simulink model "gm_FFT"  (R2025a)
settings: Solver=VariableStepAuto  StartTime=0.0  StopTime=10.0  RelTol=1e-3
libraries: dsphdlxfrm2 x1
settings Model: Creator=ivanmart  LastModifiedBy=ivanmart
settings OptimizationCC: BlockReduction=off  ConditionallyExecuteInputs=off
settings DebuggingCC: InheritedTsInSrcMsg=none

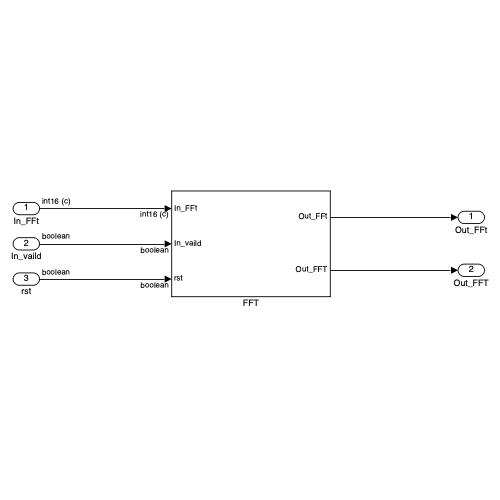
[thumbnail: Simulink's stored preview of the top-level diagram]
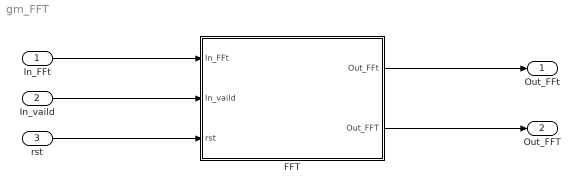
== system gm_FFT ==
  In_FFt : Inport  OutDataTypeStr=fixdt(1,16,0)
      settings: SignalType=complex
  In_vaild : Inport  Port=2  OutDataTypeStr=boolean
  rst : Inport  Port=3  OutDataTypeStr=boolean
  FFT : Subsystem
  Out_FFt : Outport
  Out_FFT : Outport  Port=2
  wires:
  FFT/2(Out_FFT) -> Out_FFT/1
  FFT/1(Out_FFt) -> Out_FFt/1
  rst/1 -> FFT/3(rst)
  In_vaild/1 -> FFT/2(In_vaild)
  In_FFt/1 -> FFT/1(In_FFt)

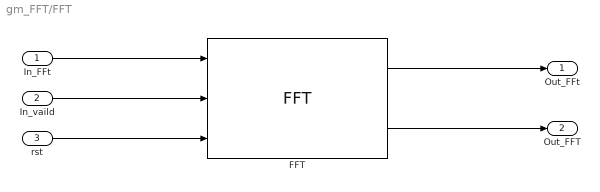
== system gm_FFT/FFT ==
  In_FFt : Inport  OutDataTypeStr=fixdt(1,16,0)
      settings: SignalType=complex
  In_vaild : Inport  Port=2  OutDataTypeStr=boolean
  rst : Inport  Port=3  OutDataTypeStr=boolean
  FFT : dsphdlxfrm2/FFT  Architecture=Streaming Radix 2^2  FFTLengthSource=Property  FFTLength=4096  FFTLengthMax=1024  ComplexMultiplication=Use 4 multipliers and 2 adders  BitReversedOutput=off  BitReversedInput=off  Normalize=off  SimulateUsing=Code generation  RoundingMethod=Floor  ResetInputPort=on  StartOutputPort=off  EndOutputPort=off
  Out_FFt : Outport
  Out_FFT : Outport  Port=2
  wires:
  In_FFt/1 -> FFT/1
  FFT/2 -> Out_FFT/1
  FFT/1 -> Out_FFt/1
  In_vaild/1 -> FFT/2
  rst/1 -> FFT/3
